simulink model "Linear_2nd_order_model4DataProduction"  (R2024b)
settings: Solver=ode3  StartTime=0.0  StopTime=max_sim_time  FixedStep=T_sample  RelTol=1e-3  EnableMultiTasking=on
values from neighbouring files (symbols this model uses):
  a = -2*kesi* wn    (= -4.2)    [Linear_2nd_order_Sys_Model4Datacollection.m]    (also in Model_parameters_Ident.m = x_model(1))
  b = K*wn^2    (= 9)    [Linear_2nd_order_Sys_Model4Datacollection.m]    (also in Model_parameters_Ident.m = x_model(3))
  base = 0    [Linear_2nd_order_Sys_Model4Datacollection.m]
  c = -wn^2    (= -9)    [Linear_2nd_order_Sys_Model4Datacollection.m]    (also in Model_parameters_Ident.m = x_model(2))
  f0 = 1    [Linear_2nd_order_Sys_Model4Datacollection.m]    (also in Model_parameters_Ident.m = x_model(4))
  fluctuation_range = 1    [Linear_2nd_order_Sys_Model4Datacollection.m]
settings Model: Creator=shaocan  LastModifiedBy=sk3547969879
settings SolverCC: AlgebraicLoopSolver=TrustRegion
settings DataIOCC: LimitDataPoints=on  SaveFormat=Array  ReturnWorkspaceOutputs=off
settings OptimizationCC: LifeSpan=inf
settings DebuggingCC: UnconnectedInputMsg=warning  UnconnectedOutputMsg=warning  UnconnectedLineMsg=warning  SFUnexpectedBacktrackingDiag=warning  SFNoUnconditionalDefaultTransitionDiag=warning  SFExecutionAtInitializationDiag=none  ArithmeticOperatorsInVariantConditions=warning
settings HardwareCC: ProdBitPerPointer=32  ProdBitPerSizeT=32  ProdBitPerPtrDiffT=32  ProdLargestAtomicFloat=None  ProdIntDivRoundTo=Undefined  ProdEndianess=Unspecified  ProdWordSize=32  ProdHWDeviceType=32-bit Generic
settings ModelReferenceCC: EnableRefExpFcnMdlSchedulingChecks=on  PropagateSignalLabelsOutOfModel=off
settings SFSimCC: SimUseLocalCustomCode=off  CustomCodeUndefinedFunction=UseInterfaceOnly
settings RTWCC: RTWUseLocalCustomCode=off  GPUComputeCapability=3.5  DLArmComputeVersion=19.05
settings CodeAppCC: StateflowObjectComments=on
settings GRTTargetCC: TargetLangStandard=C89/C90 (ANSI)
settings ConfigComp: CovMetricSettings=dw  CovSaveCumulativeToWorkspaceVar=on  CovSaveSingleToWorkspaceVar=on  CovExternalEMLEnable=off  CovSFcnEnable=off

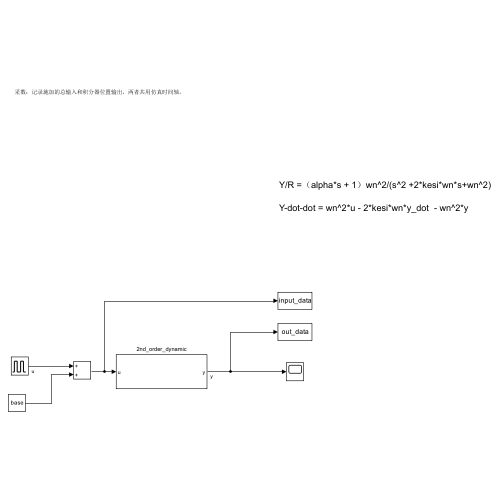
[thumbnail: Simulink's stored preview of the top-level diagram]
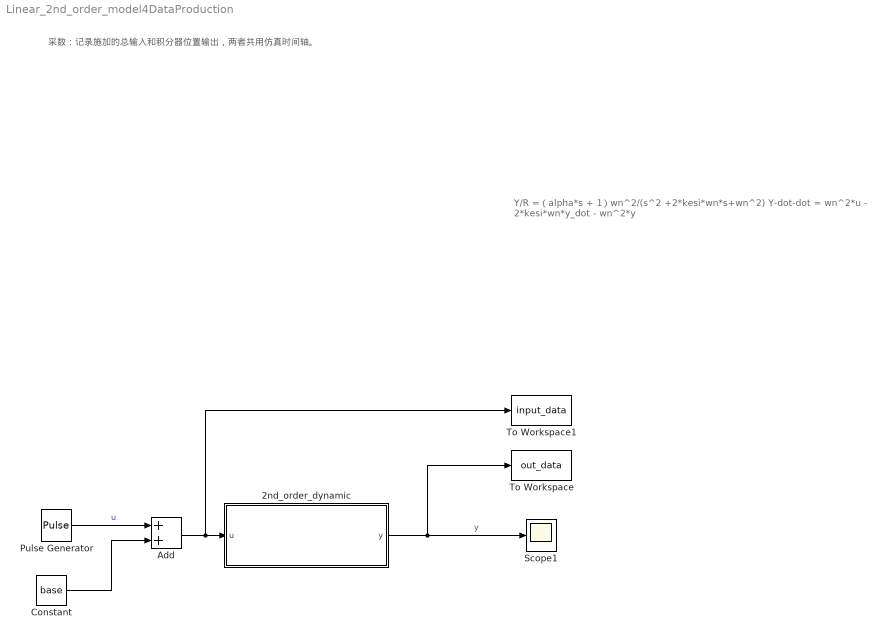
== system Linear_2nd_order_model4DataProduction ==
  note: Y/R =（alpha*s + 1）wn^2/(s^2 +2*kesi*wn*s+wn^2)
      |
      | Y-dot-dot = wn^2*u - 2*kesi*wn*y_dot - wn^2*y
  note: 采数：记录施加的总输入和积分器位置输出，两者共用仿真时间轴。
  2nd_order_dynamic : Subsystem
  Add : Sum
  Constant : Constant  Value=base
  Pulse Generator : DiscretePulseGenerator  PulseType=Time based  Amplitude=fluctuation_range  Period=5  PulseWidth=50
  Scope1 : Scope
  To Workspace : ToWorkspace  VariableName=out_data  SaveFormat=Timeseries  SampleTime=-1
  To Workspace1 : ToWorkspace  VariableName=input_data  SaveFormat=Timeseries  SampleTime=-1
  wires:
  Pulse Generator/1 -> Add/1  "u"
  2nd_order_dynamic/1(y) -> Scope1/1, To Workspace/1  "y"
  Add/1 -> To Workspace1/1, 2nd_order_dynamic/1(u)
  Constant/1 -> Add/2

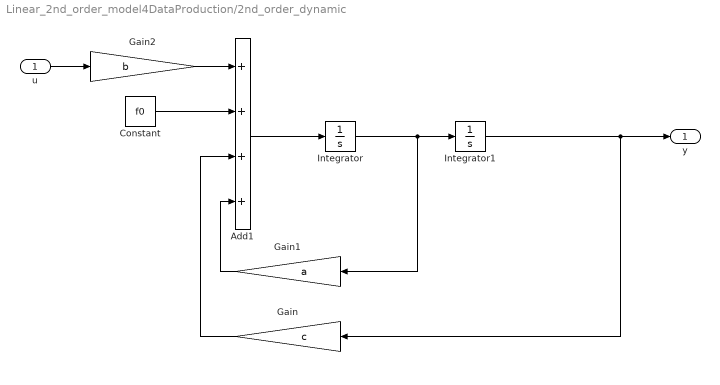
== system Linear_2nd_order_model4DataProduction/2nd_order_dynamic ==
  u : Inport
  Add1 : Sum  Inputs=++++
  Constant : Constant  Value=f0
  Gain : Gain  Gain=c
  Gain1 : Gain  Gain=a
  Gain2 : Gain  Gain=b
  Integrator : Integrator
  Integrator1 : Integrator
  y : Outport
  wires:
  Add1/1 -> Integrator/1
  Gain/1 -> Add1/3
  u/1 -> Gain2/1
  Integrator/1 -> Gain1/1, Integrator1/1
  Integrator1/1 -> Gain/1, y/1
  Gain2/1 -> Add1/1
  Gain1/1 -> Add1/4
  Constant/1 -> Add1/2
